simulink subsystem "BatteryEq"  (R2025b)
settings: Solver=VariableStepAuto  StartTime=0.0  StopTime=10.0  RelTol=1e-3
undefined symbols (not defined in the file or in its folder): battery
libraries: fl_lib x4, nesl_utility x3, batteryecm_lib x1, simulink x1
settings Model: Creator=jjha  LastModifiedBy=jjha

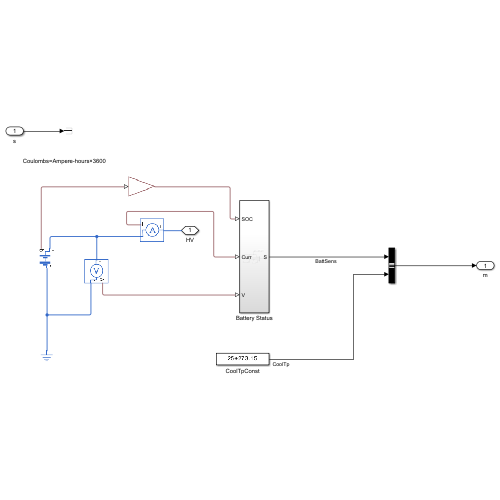
[thumbnail: Simulink's stored preview of the top-level diagram]
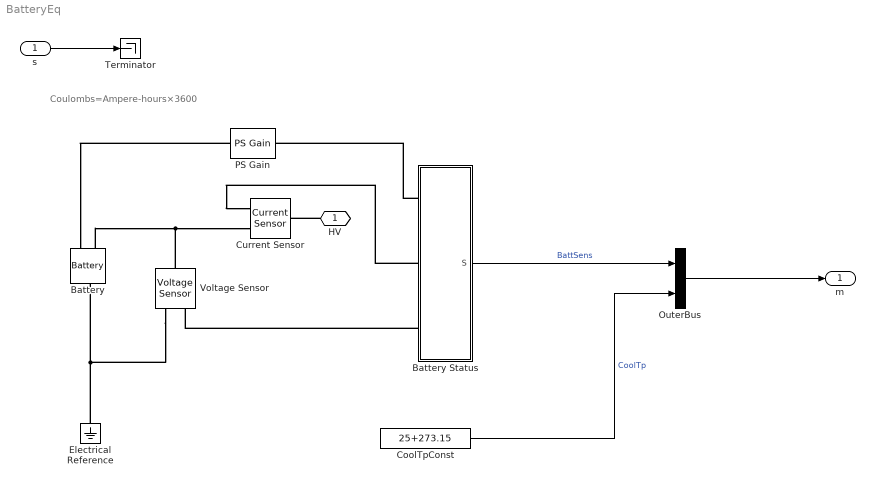
== system BatteryEq ==
  note: Coulombs=Ampere-hours×3600
  s : Inport
  Battery : batteryecm_lib/Battery  Vnom=battery.Vnom V  prm_dir=simscape.enum.battery.prm_dir.disabled  R1_dis=2 Ohm  R1_ch=2 Ohm  R1=battery.R1*battery.Ns/battery.Np mOhm  prm_AH=simscape.enum.battery.prm_AH.finite  AH=battery.AH A*hr  V1=battery.V1 V  AH1=battery.AH1 A*hr  prm_R2=simscape.enum.battery.prm_R2.disabled  R2=2000 Ohm  Tmeas=298.15 K  charge_measurement_port=simscape.enum.battery.enable.yes  prm_dyn=simscape.enum.battery.prm_dyn.off  Rp1=0.005 Ohm  tau1=30 s  Rp2=0.005 Ohm  tau2=30 s  Rp3=0.005 Ohm  tau3=30 s  Rp4=0.005 Ohm  tau4=30 s  Rp5=0.005 Ohm  tau5=30 s  prm_fade=simscape.enum.battery.prm_fade.disabled  N_fade=100  AH_fade=45 A*hr  R1_fade=2.02 Ohm  R1_ch_fade=2.02 Ohm  V1_fade=10.35 V  prm_age=simscape.enum.battery.prm_age.disabled  prm_age_OCV=simscape.enum.battery.prm_age_OCV.OCV  OCV_age=0.9  SOC_age=60  Tmeas_age=298.15 K  delta_time_age_vec=[0] d  temperature_age_vec=[273] K  OCV_scaling_age=2.2134e6  OCV_offset_age=1.632e6  temp_exp_age=0.515833569 V  t_exp_age=0.75  Vnom_T2=12 V  R1_T2=2.2 Ohm  R1_T2_dis=2.2 Ohm  R1_T2_ch=2.2 Ohm  V1_T2=11.4 V  R2_T2=2200 Ohm  Rp1_T2=0.005 Ohm  tau1_T2=30 s  Rp2_T2=0.005 Ohm  tau2_T2=30 s  Rp3_T2=0.005 Ohm  tau3_T2=30 s  Rp4_T2=0.005 Ohm  tau4_T2=30 s  Rp5_T2=0.005 Ohm  tau5_T2=30 s  Tmeas2=273.15 K  thermal_port=simscape.enum.thermaleffects.omit  thermal_mass=30000 J/K  i_specify=off  i_priority=High  i=0 A  i_nominal_specify=off  i_nominal_value=1  i_nominal_unit=A  v_specify=off  v_priority=None  v=0 V  v_nominal_specify=off  v_nominal_value=1  v_nominal_unit=V  charge_specify=on  charge_priority=High  charge=battery.AH *battery.initialPackSOC A*hr  charge_nominal_specify=off  charge_nominal_value=1  charge_nominal_unit=A*hr  num_cycles_specify=off  num_cycles_priority=High  num_cycles=0  num_cycles_nominal_specify=off  num_cycles_nominal_value=1  num_cycles_nominal_unit=1  temperature_specify=off  temperature_priority=High  temperature=298.15 K  temperature_nominal_specify=off  temperature_nominal_value=1  temperature_nominal_unit=K
      settings: InternalSimscapePortConfiguration="{\"Bottom\":[],\"Left\":[{\"id\":\"p\",\"label\":\"+\",\"type\":\"foundation.electrical.electrical\"},{\"id\":\"q\",\"label\":\"q\",\"type\":\"output\"}],\"Right\":[{\"id\":\"n\",\"label\":\"-\",\"type\":\"foundation.electrical.electrical\"}],\"Top\":[]}"
  Battery Status : Subsystem
  CoolTpConst : Constant  Value=25+273.15  OutDataTypeStr=double
  Current Sensor : fl_lib/Electrical/Electrical Sensors/Current Sensor
  Electrical Reference : fl_lib/Electrical/Electrical Elements/Electrical Reference
  OuterBus : BusCreator  Inputs=2
  PS Gain : fl_lib/Physical Signals/Functions/PS Gain  gain=1/(3600*battery.AH)
  Terminator : Terminator
  Voltage Sensor : fl_lib/Electrical/Electrical Sensors/Voltage Sensor
  HV : PMIOPort  Side=Right
  m : Outport
  wires:
  s/1 -> Terminator/1
  OuterBus/1 -> m/1
  CoolTpConst/1 -> OuterBus/2  "CoolTp"
  Battery Status/1(S) -> OuterBus/1  "BattSens"
  connections:
  Voltage Sensor/RConn2 -- Electrical Reference/LConn1 -- Battery/RConn1
  Voltage Sensor/LConn1 -- Current Sensor/RConn2 -- Battery/LConn1
  HV/RConn1 -- Current Sensor/LConn1
  PS Gain/LConn1 -- Battery/LConn2
  Battery Status/LConn2 -- Current Sensor/RConn1
  Battery Status/LConn1 -- PS Gain/RConn1
  Battery Status/LConn3 -- Voltage Sensor/RConn1

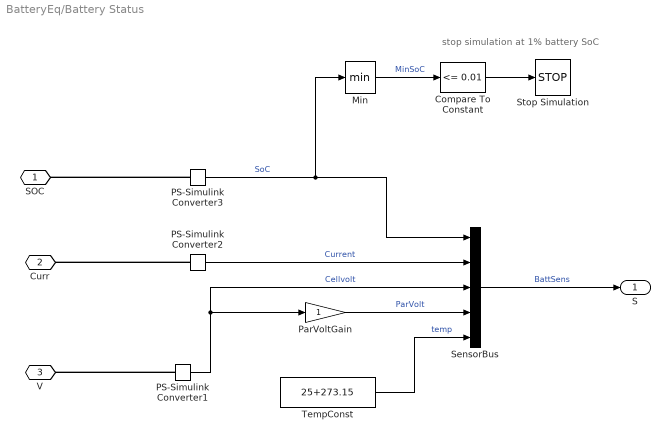
== system BatteryEq/Battery Status ==
  note: stop simulation at 1% battery SoC
  Compare To Constant : simulink/Logic and Bit Operations/Compare To Constant  relop=<=  const=0.01  OutDataTypeStr=boolean
  Min : MinMax
  PS-Simulink Converter1 : nesl_utility/PS-Simulink Converter  PhysicalDomain=network_engine_domain  SubClassName=ps_output  LeftPortType=input  RightPortType=output  PseudoPeriodic=off  Frequencies=[]  VectorFormat=inherit  Unit=V  AffineConversion=off
  PS-Simulink Converter2 : nesl_utility/PS-Simulink Converter  PhysicalDomain=network_engine_domain  SubClassName=ps_output  LeftPortType=input  RightPortType=output  PseudoPeriodic=off  Frequencies=[]  VectorFormat=inherit  Unit=inherit  AffineConversion=off
  PS-Simulink Converter3 : nesl_utility/PS-Simulink Converter  PhysicalDomain=network_engine_domain  SubClassName=ps_output  LeftPortType=input  RightPortType=output  PseudoPeriodic=off  Frequencies=[]  VectorFormat=inherit  Unit=inherit  AffineConversion=off
  ParVoltGain : Gain
  SensorBus : BusCreator  Inputs=5
  Stop Simulation : Stop
  TempConst : Constant  Value=25+273.15  OutDataTypeStr=double
  SOC : PMIOPort  Side=Left
  Curr : PMIOPort  Port=2  Side=Left
  V : PMIOPort  Port=3  Side=Left
  S : Outport
  wires:
  SensorBus/1 -> S/1  "BattSens"
  Min/1 -> Compare To Constant/1  "MinSoC"
  ParVoltGain/1 -> SensorBus/4  "ParVolt"
  Compare To Constant/1 -> Stop Simulation/1
  PS-Simulink Converter1/1 -> SensorBus/3, ParVoltGain/1  "Cellvolt"
  TempConst/1 -> SensorBus/5  "temp"
  PS-Simulink Converter2/1 -> SensorBus/2  "Current"
  PS-Simulink Converter3/1 -> SensorBus/1, Min/1  "SoC"
  connections:
  PS-Simulink Converter2/LConn1 -- Curr/RConn1
  PS-Simulink Converter1/LConn1 -- V/RConn1
  PS-Simulink Converter3/LConn1 -- SOC/RConn1
